simulink library "three_phase_pwm_modulator"  (R2025b)
settings: Solver=VariableStepAuto  StartTime=0.0  StopTime=10.0  RelTol=1e-3
undefined symbols (not defined in the file): dead_time_INV, fPWM_INV, tc
libraries: single_phase_pwm_modulator x1
settings Model: Creator=dbagn  LastModifiedBy=dbagn

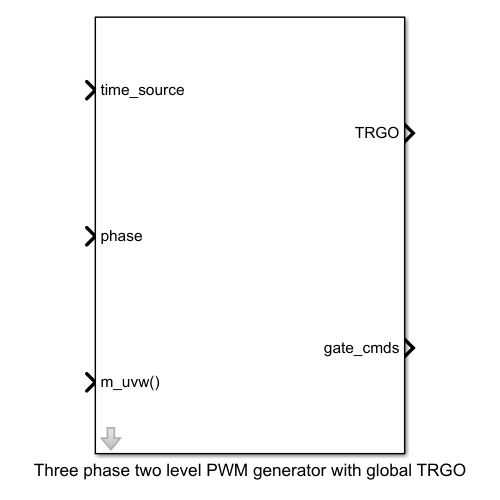
[thumbnail: Simulink's stored preview of the top-level diagram]
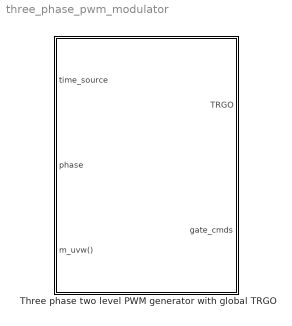
== system three_phase_pwm_modulator ==
  Three phase two level PWM generator with global TRGO : Subsystem  mask{f=fPWM_INV, m_up=0.98, m_low=0.02, dead_time=dead_time_INV, pos_cmd_gate=15, neg_cmd_gate=-10, polarity=1, tc=tc, double_sampling=1}
      mask prompts: f "Frequency (Hz)"; m_up "Max Input Modulation Value"; m_low "Min Input Modulation Value"; dead_time "Dead Time (s)"; pos_cmd_gate "Positive Gate Voltage (V)"; neg_cmd_gate "Negative Gate Voltage (V)"; polarity "Polarity (pu)"; tc "Sampling time"

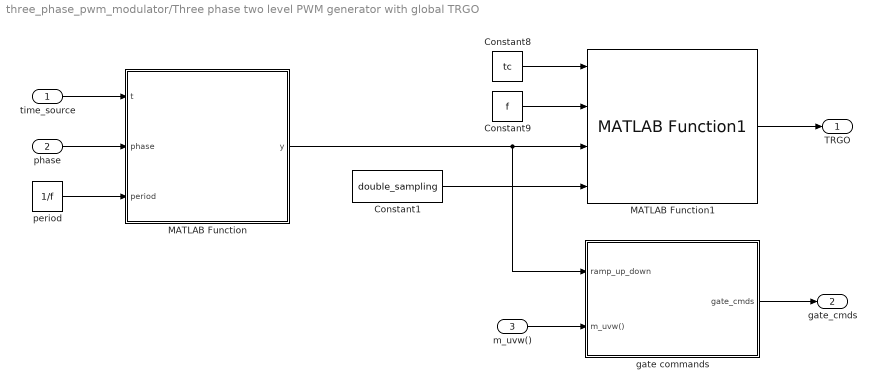
== system three_phase_pwm_modulator/Three phase two level PWM generator with global TRGO ==
  time_source : Inport
  phase : Inport  Port=2
  m_uvw() : Inport  Port=3
  Constant1 : Constant  Value=double_sampling
  Constant8 : Constant  Value=tc
  Constant9 : Constant  Value=f
  MATLAB Function : MATLAB Function  TreatAsAtomicUnit=on  SystemSampleTime=tc
  MATLAB Function1 : single_phase_pwm_modulator/Single phase two level PWM generator with global TRGO/MATLAB Function1  SystemSampleTime=tc  VariantActivationTime=update diagram  EmptyChoice=off  PassThrough=off  PassThroughVariantControl=(default)  EmptyChoiceVariantControl=(default)  AllowFlexibleInterface=on  Latency=0  AutoFrameSizeCalculation=off
  gate commands : Subsystem
  period : Constant  Value=1/f
  TRGO : Outport
  gate_cmds : Outport  Port=2
  wires:
  period/1 -> MATLAB Function/3(period)
  phase/1 -> MATLAB Function/2(phase)
  MATLAB Function/1(y) -> gate commands/1(ramp_up_down), MATLAB Function1/3
  MATLAB Function1/1 -> TRGO/1
  Constant8/1 -> MATLAB Function1/1
  Constant9/1 -> MATLAB Function1/2
  m_uvw()/1 -> gate commands/2(m_uvw())
  gate commands/1(gate_cmds) -> gate_cmds/1
  time_source/1 -> MATLAB Function/1(t)
  Constant1/1 -> MATLAB Function1/4

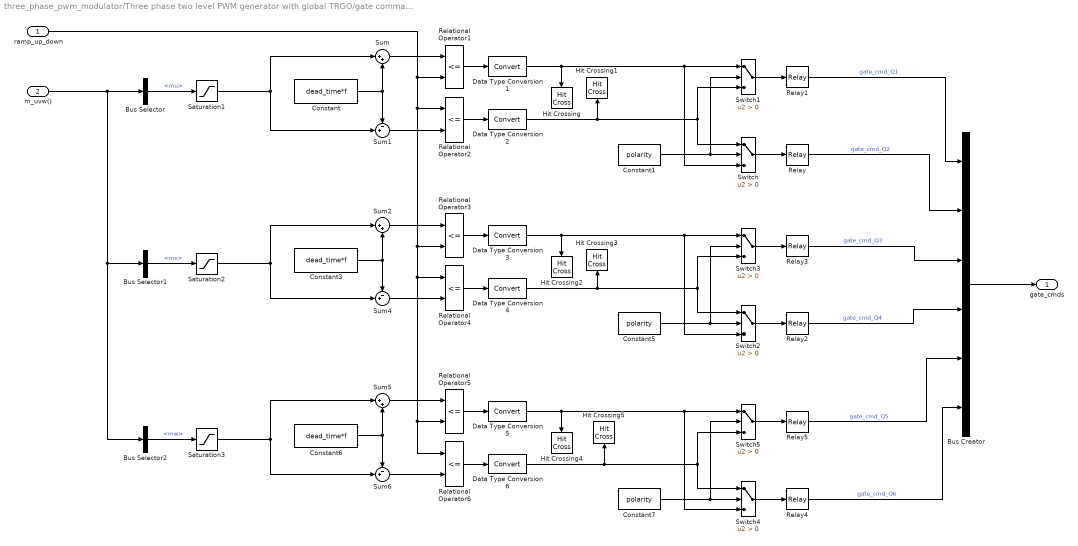
== system three_phase_pwm_modulator/Three phase two level PWM generator with global TRGO/gate commands ==
  ramp_up_down : Inport
  m_uvw() : Inport  Port=2
  Bus Creator : BusCreator  Inputs=6
  Bus Selector : BusSelector  OutputSignals=mu
  Bus Selector1 : BusSelector  OutputSignals=mv
  Bus Selector2 : BusSelector  OutputSignals=mw
  Constant : Constant  Value=dead_time*f
  Constant1 : Constant  Value=polarity
  Constant3 : Constant  Value=dead_time*f
  Constant5 : Constant  Value=polarity
  Constant6 : Constant  Value=dead_time*f
  Constant7 : Constant  Value=polarity
  Data Type Conversion{1..6} (6 alike) : DataTypeConversion
  Hit Crossing{,1..5} (6 alike) : HitCross  ShowOutputPort=off
  Relational Operator{1..6} (6 alike) : RelationalOperator  Operator=<=  InputSameDT=off
  Relay{,1..5} (6 alike) : Relay  OnOutputValue=pos_cmd_gate  OffOutputValue=neg_cmd_gate
  Saturation1 : Saturate  UpperLimit=m_up  LowerLimit=m_low
  Saturation2 : Saturate  UpperLimit=m_up  LowerLimit=m_low
  Saturation3 : Saturate  UpperLimit=m_up  LowerLimit=m_low
  Sum : Sum  Inputs=|++  SaturateOnIntegerOverflow=on
  Sum1 : Sum  Inputs=-+|  SaturateOnIntegerOverflow=on
  Sum2 : Sum  Inputs=|++  SaturateOnIntegerOverflow=on
  Sum4 : Sum  Inputs=-+|  SaturateOnIntegerOverflow=on
  Sum5 : Sum  Inputs=|++  SaturateOnIntegerOverflow=on
  Sum6 : Sum  Inputs=-+|  SaturateOnIntegerOverflow=on
  Switch{,1..5} (6 alike) : Switch  Criteria=u2 > Threshold  SaturateOnIntegerOverflow=off  InputSameDT=off
  gate_cmds : Outport
  wires:
  Data Type Conversion6/1 -> Switch4/1, Switch5/3, Hit Crossing5/1
  Constant1/1 -> Switch1/2, Switch/2
  Data Type Conversion1/1 -> Switch/3, Switch1/1, Hit Crossing/1
  Constant3/1 -> Sum4/1, Sum2/2
  m_uvw()/1 -> Bus Selector2/1, Bus Selector1/1, Bus Selector/1
  Relay4/1 -> Bus Creator/6  "gate_cmd_Q6"
  Constant6/1 -> Sum5/2, Sum6/1
  Saturation1/1 -> Sum1/2, Sum/1
  Data Type Conversion3/1 -> Switch2/3, Switch3/1, Hit Crossing2/1
  Data Type Conversion2/1 -> Switch/1, Switch1/3, Hit Crossing1/1
  Relational Operator1/1 -> Data Type Conversion1/1
  Bus Creator/1 -> gate_cmds/1
  Data Type Conversion5/1 -> Switch4/3, Switch5/1, Hit Crossing4/1
  Sum1/1 -> Relational Operator2/2
  Constant5/1 -> Switch2/2, Switch3/2
  Switch/1 -> Relay/1
  Sum/1 -> Relational Operator1/1
  Relational Operator6/1 -> Data Type Conversion6/1
  Relay2/1 -> Bus Creator/4  "gate_cmd_Q4"
  Saturation3/1 -> Sum5/1, Sum6/2
  Constant7/1 -> Switch5/2, Switch4/2
  Sum5/1 -> Relational Operator5/1
  Bus Selector/1 -> Saturation1/1  "<mu>"
  Data Type Conversion4/1 -> Switch2/1, Switch3/3, Hit Crossing3/1
  ramp_up_down/1 -> Relational Operator3/2, Relational Operator6/1, Relational Operator5/2, Relational Operator4/1, Relational Operator2/1, Relational Operator1/2
  Switch4/1 -> Relay4/1
  Relational Operator5/1 -> Data Type Conversion5/1
  Switch5/1 -> Relay5/1
  Saturation2/1 -> Sum4/2, Sum2/1
  Relational Operator3/1 -> Data Type Conversion3/1
  Sum2/1 -> Relational Operator3/1
  Switch1/1 -> Relay1/1
  Relay3/1 -> Bus Creator/3  "gate_cmd_Q3"
  Relational Operator2/1 -> Data Type Conversion2/1
  Bus Selector1/1 -> Saturation2/1  "<mv>"
  Switch3/1 -> Relay3/1
  Sum4/1 -> Relational Operator4/2
  Relay/1 -> Bus Creator/2  "gate_cmd_Q2"
  Relational Operator4/1 -> Data Type Conversion4/1
  Bus Selector2/1 -> Saturation3/1  "<mw>"
  Relay1/1 -> Bus Creator/1  "gate_cmd_Q1"
  Sum6/1 -> Relational Operator6/2
  Constant/1 -> Sum/2, Sum1/1
  Relay5/1 -> Bus Creator/5  "gate_cmd_Q5"
  Switch2/1 -> Relay2/1

== matlab function three_phase_pwm_modulator/Three phase two level PWM generator with global TRGO/MATLAB Function ==
  data: t input; y output; phase input; period input
function y = ramp_up_down(t,phase,period)
x = sin(2*pi/period*t - phase -pi/2);
y = asin(x)/pi + 1/2;
